simulink model "Full_Wave_Rectifier"  (R2024b)
settings: Solver=VariableStepAuto  StartTime=0.0  StopTime=0.1  RelTol=1e-3
libraries: fl_lib x10, nesl_utility x3
settings Model: Creator=HP  LastModifiedBy=HP

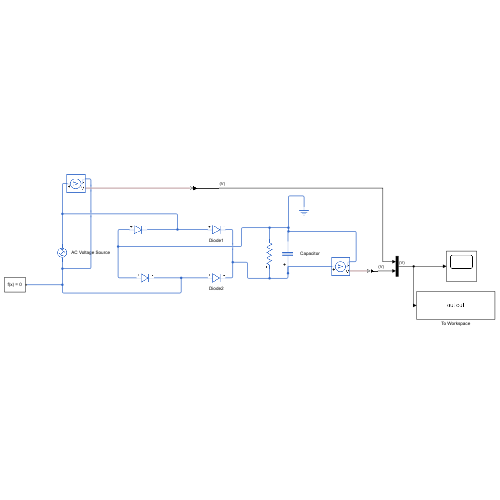
[thumbnail: Simulink's stored preview of the top-level diagram]
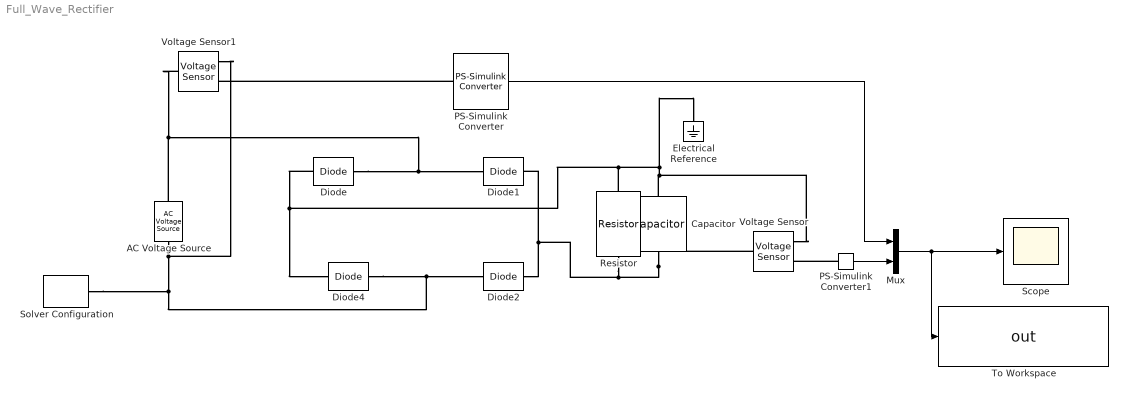
== system Full_Wave_Rectifier ==
  AC Voltage Source : fl_lib/Electrical/Electrical Sources/AC Voltage Source  amp=10 V  shift=0 deg  frequency=50 Hz
  Capacitor : fl_lib/Electrical/Electrical Elements/Capacitor  c=100e-6 F  r=1e-6 Ohm  g=0 1/Ohm  i_specify=off  i_priority=None  i=0 A  i_nominal_specify=off  i_nominal_value=1  i_nominal_unit=A  v_specify=off  v_priority=None  v=0 V  v_nominal_specify=off  v_nominal_value=1  v_nominal_unit=V  vc_specify=off  vc_priority=High  vc=0 V  vc_nominal_specify=off  vc_nominal_value=1  vc_nominal_unit=V
  Diode{,1..2,4} (4 alike) : fl_lib/Electrical/Electrical Elements/Diode  Vf=0.6 V  Ron=0.3 Ohm  Goff=1e-8 1/Ohm  i_specify=off  i_priority=None  i=0 A  i_nominal_specify=off  i_nominal_value=1  i_nominal_unit=A  v_specify=off  v_priority=None  v=0 V  v_nominal_specify=off  v_nominal_value=1  v_nominal_unit=V
  Electrical Reference : fl_lib/Electrical/Electrical Elements/Electrical Reference
  Mux : Mux  Inputs=2
  PS-Simulink Converter : nesl_utility/PS-Simulink Converter  PhysicalDomain=network_engine_domain  SubClassName=ps_output  LeftPortType=input  RightPortType=output  PseudoPeriodic=off  Frequencies=[]  VectorFormat=inherit  Unit=inherit  AffineConversion=off
  PS-Simulink Converter1 : nesl_utility/PS-Simulink Converter  PhysicalDomain=network_engine_domain  SubClassName=ps_output  LeftPortType=input  RightPortType=output  PseudoPeriodic=off  Frequencies=[]  VectorFormat=inherit  Unit=inherit  AffineConversion=off
  Resistor : fl_lib/Electrical/Electrical Elements/Resistor  R=100 Ohm  i_specify=off  i_priority=None  i=0 A  i_nominal_specify=off  i_nominal_value=1  i_nominal_unit=A  v_specify=off  v_priority=None  v=0 V  v_nominal_specify=off  v_nominal_value=1  v_nominal_unit=V
  Scope : Scope
  Solver Configuration : nesl_utility/Solver Configuration  PhysicalDomain=network_engine_domain  SubClassName=solver  LeftPortType=input  RightPortType=generic  Tones=[]  Harmonics=[]  SimulateNoise=off  Profile=off  UseLocalSampling=off  EnableSwitchedLinearOptims=on  FrequencyDomain=off  UseCCode=off  RelTol=0.001  AbsTol=0.001  MinStep=1e-09  ToWorkspace=off  RevertToSquareIcSolve=off  NumHomotopyIterations=100  PhasorMode=off  PhasorModeNumHarmonics=1  ConsistencySolver=NEWTON_XTOL_AFTER_FTOL  IndexReductionMethod=DerivativeReplacement  DoDC=off  ResidualTolerance=1e-09  ConsistencyTolSource=GLOBAL  ConsistencyAbsTol=0.001  ConsistencyRelTol=0.001  ConsistencyTolFactor=0.001  UseLocalSolver=off  LocalSolverChoice=NE_BACKWARD_EULER_ADVANCER  ResolveIndetEquations=on  FunctionEvalNumThread=1  LocalSolverSampleTime=0.001  DoFixedCost=off  MaxNonlinIter=3  MaxModeIter=2  ComputeImpulses=off  ImpulseIterations=2  LinearAlgebra=auto  LinearAlgebraNumThread=0  EquationFormulation=NE_TIME_EF  DelaysMemoryBudget=1024  AutomaticFiltering=on  FilteringTimeConstant=0.001  PartitionStorageMethod=AS_NEEDED  PartitionMemoryBudget=1024  PartitionMethod=ROBUST  MultibodyUseLocalSolver=off  MultibodyLocalSolverChoice=ODE1  MultibodyLocalSolverSampleTime=0.001
  To Workspace : ToWorkspace  VariableName=out  SaveFormat=Timeseries  SampleTime=-1
  Voltage Sensor : fl_lib/Electrical/Electrical Sensors/Voltage Sensor
  Voltage Sensor1 : fl_lib/Electrical/Electrical Sensors/Voltage Sensor
  wires:
  PS-Simulink Converter1/1 -> Mux/2
  PS-Simulink Converter/1 -> Mux/1
  Mux/1 -> Scope/1, To Workspace/1
  connections:
  Diode/RConn1 -- Voltage Sensor1/LConn1 -- AC Voltage Source/LConn1 -- Diode1/LConn1
  Diode4/RConn1 -- Voltage Sensor1/RConn2 -- AC Voltage Source/RConn1 -- Solver Configuration/RConn1 -- Diode2/LConn1
  Diode/LConn1 -- Voltage Sensor/RConn2 -- Capacitor/RConn1 -- Electrical Reference/LConn1 -- Resistor/RConn1 -- Diode4/LConn1
  Diode2/RConn1 -- Voltage Sensor/LConn1 -- Capacitor/LConn1 -- Resistor/LConn1 -- Diode1/RConn1
  PS-Simulink Converter/LConn1 -- Voltage Sensor1/RConn1
  PS-Simulink Converter1/LConn1 -- Voltage Sensor/RConn1
